simulink model "YMBOX_Control_Core"  (R2024b)
settings: Solver=FixedStepDiscrete  StartTime=0.0  StopTime=3  RelTol=1e-3
PreLoadFcn:
  | run(fullfile(fileparts(get_param(bdroot,'FileName')), 'YMBOX_Deluxe_init.m'));
InitFcn:
  | YMBOX_InitializeModel('core',bdroot);
model workspace (MAT data in the model file):
  KuMDAS_ObserverBuildVariant : Simulink.Parameter (value not decoded)
undefined symbols (not defined in the file or in its folder): CeMDSM_DrvModeIfStart_enum, CeMDSM_DrvModeSpdSens_enum, CeMDSM_DrvModeSpdSmo_enum, CeMDSM_DrvModeTrq_enum, Cf_CONTROL_TASK_TIME_S, KbMDAS_SmoDeadTimeCompEnable_flg, KbMDSA_ActiveInverterCompEnable_flg, KbMDSA_UnifiedVoltageLimitEnable_flg, KbMDSP_DCBusVoltReportFilterEnable_flg, KbMDTM_DAxisPriorityInFW_flg, KbMDTM_FieldWeakeningEnable_flg, KbMDTM_FinalIqAntiWindupEnable_flg, KbMDTM_SensorlessFieldWeakeningEnable_flg, KbMDTM_TorquePriorityBelowBase_flg, KbMDTM_UnifiedConstraintEnable_flg, KfMDAS_ControlCountToElecRad_NULL, KfMDAS_IfAccel_rpms, KfMDAS_IfAlignTime_s, KfMDAS_IfBlendTime_s, KfMDAS_IfSwitchSpd_rpm, KfMDAS_NativeCountToMechRad_NULL, KfMDAS_ObserverExitRatio_NULL, KfMDAS_SlsCtrlPeriod_s, KfMDAS_SlsEAngleInit_rad, KfMDAS_SlsElecSpdMax_rads, KfMDAS_SlsElecSpdMin_rads, KfMDAS_SlsTwoPi_rad, KfMDAS_SmoAngleOffset_rad, KfMDAS_SmoCurrentZohCoefA_NULL, KfMDAS_SmoCurrentZohCoefB_AperV, KfMDAS_SmoDeadTimeCurrentBoundary_A, KfMDAS_SmoDeadTimeDuty_NULL, KfMDAS_SmoDeadTimePolarity_NULL, KfMDAS_SmoDeviceDrop_V, KfMDAS_SmoEmfLpfCoefA_NULL, KfMDAS_SmoEmfLpfCoefB_NULL, KfMDAS_SmoEmfLpfInvPole_s, KfMDAS_SmoErrBoundaryMax_A, KfMDAS_SmoErrBoundarySpan_A, KfMDAS_SmoGainSchedAlpha_NULL, KfMDAS_SmoGainSchedAngleComp_rad, KfMDAS_SmoGainSchedEmfLow_V, KfMDAS_SmoGainSchedInvSpan_PerV, KfMDAS_SmoLdMinusLq_H, KfMDAS_SmoPllKiTs_NULL, KfMDAS_SmoPllKp_NULL, KfMDAS_SmoPllMinEmf_V, KfMDAS_SmoPllSpeedLpfAlpha_NULL, KfMDAS_SmoSlideGainMin_V, KfMDAS_SmoSlideGainSpan_V, KfMDAS_SmoSwitchSpd_rpm, KfMDAS_SmoTotalDelay_s, KfMDCC_DqSoftwareOverCurrentThreshold_A, KfMDCC_PiKcTsId_NULL, KfMDCC_PiKcTsIq_NULL, KfMDCC_PiKiTsId_NULL, KfMDCC_PiKiTsIq_NULL, KfMDCC_PiKpValueId_NULL, KfMDCC_PiKpValueIq_NULL, KfMDCC_PwmFreq_Hz ... (+84)
libraries: YMBOX_SharedMath_Lib x11, spsabctoAlphaBetaZeroLib x1
(part 2 of 8)

== system YMBOX_Control_Core/MDSP ==
  MINP_outputs : Inport  OutDataTypeStr=Bus: MINP_output
  MDSA_outputs : Inport  Port=2  OutDataTypeStr=Bus: MDSA_output
  trig_MDSP_ControlTask : TriggerPort  TriggerType=function-call  VariantControl=(inherit)
  DCBusCurrentFilterState : UnitDelay  InitialCondition=single(0)  SampleTime=-1
  DCBusCurrentInvalidHold : Switch  Threshold=0.5
  DCBusCurrentMean4 : MATLABSystem  System=dsp.simulink.MovingAverage  Method=Sliding window  ForgettingFactorPort=off  SpecifyWindowLength=on  WindowLength=KfMDSP_DCBusCurAvgWindow_cnt  OverlapLength=KfMDSP_DCBusCurAvgWindow_cnt-1  AllowArbitraryInputLength=off  ForgettingFactor=0.9  SimulateUsing=Code generation
      mask Type: dsp.simulink.MovingAverage
      mask Display: disp(['Moving' char(10) 'Average']);
  DCBus_Current_Source_Variant : Subsystem  Variant=on
  DCBus_Voltage_Filter : Subsystem
  Direct_Input_Selector : BusSelector  OutputSignals=VMIN_Dir_UCurSenrCurDet_A,VMIN_Dir_VCurSenrCurDet_A,VMIN_Dir_WCurSenrCurDet_A,VMIN_Dir_UCurSenrCurErr_NULL,VMIN_Dir_VCurSenrCurErr_NULL,VMIN_Dir_WCurSenrCurErr_NULL
  MDSP_Output_Bus : BusCreator  Inputs=13  OutDataTypeStr=Bus: MDSP_output  NonVirtualBus=on
      settings: InheritFromInputs=off
  MINP_Input_Selector : BusSelector  OutputSignals=Direct_Output,VuMINP_ResolverPositionRaw_NULL,VfMINP_DCBusVoltRaw_V
  MINP_Input_Selector1 : BusSelector  OutputSignals=VfMINP_DCBusCurPhysical_A
  PhaseSampleErrorAny : Logic  Operator=OR  Inputs=3
  PhaseSamplesValid : Logic  Operator=NOT  Inputs=1
  Phase_Current_Conditioning : Subsystem
  Previous_PWM_Selector : BusSelector  OutputSignals=VfMDSA_PwmDutyCyclePhaseU_NULL,VfMDSA_PwmDutyCyclePhaseV_NULL,VfMDSA_PwmDutyCyclePhaseW_NULL
  Resolver_Processing : Subsystem
  MDSP_outputs : Outport  OutDataTypeStr=Bus: MDSP_output
  wires:
  Direct_Input_Selector/2 -> DCBus_Current_Source_Variant/6(phaseV_A), Phase_Current_Conditioning/2(phaseV_A)  "<VMIN_Dir_VCurSenrCurDet_A>"
  Previous_PWM_Selector/2 -> DCBus_Current_Source_Variant/3(dutyV_NULL)  "<VfMDSA_PwmDutyCyclePhaseV_NULL>"
  Resolver_Processing/1(Resolver_Output) -> MDSP_Output_Bus/2  "Resolver_Output"
  DCBus_Voltage_Filter/3(VfMDSP_DCBusVoltReport_V) -> MDSP_Output_Bus/6  "VfMDSP_DCBusVoltReport_V"
  MDSP_Output_Bus/1 -> MDSP_outputs/1  "MDSP_output"
  MINP_Input_Selector/3 -> DCBus_Voltage_Filter/1(VfMINP_DCBusVoltRaw_V)  "<VfMINP_DCBusVoltRaw_V>"
  MINP_Input_Selector/2 -> Resolver_Processing/1(VuMINP_ResolverPositionRaw_NULL)  "<VuMINP_ResolverPositionRaw_NULL>"
  Direct_Input_Selector/1 -> DCBus_Current_Source_Variant/5(phaseU_A), Phase_Current_Conditioning/1(phaseU_A)  "<VMIN_Dir_UCurSenrCurDet_A>"
  Previous_PWM_Selector/3 -> DCBus_Current_Source_Variant/4(dutyW_NULL)  "<VfMDSA_PwmDutyCyclePhaseW_NULL>"
  Direct_Input_Selector/3 -> Phase_Current_Conditioning/3(phaseW_A), DCBus_Current_Source_Variant/7(phaseW_A)  "<VMIN_Dir_WCurSenrCurDet_A>"
  Direct_Input_Selector/4 -> Phase_Current_Conditioning/4(phaseUError_flg), PhaseSampleErrorAny/1  "<VMIN_Dir_UCurSenrCurErr_NULL>"
  Direct_Input_Selector/5 -> Phase_Current_Conditioning/5(phaseVError_flg), PhaseSampleErrorAny/2  "<VMIN_Dir_VCurSenrCurErr_NULL>"
  Direct_Input_Selector/6 -> Phase_Current_Conditioning/6(phaseWError_flg), PhaseSampleErrorAny/3  "<VMIN_Dir_WCurSenrCurErr_NULL>"
  MDSA_outputs/1 -> Previous_PWM_Selector/1
  PhaseSampleErrorAny/1 -> PhaseSamplesValid/1
  Previous_PWM_Selector/1 -> DCBus_Current_Source_Variant/2(dutyU_NULL)  "<VfMDSA_PwmDutyCyclePhaseU_NULL>"
  DCBus_Current_Source_Variant/2(currentValid_flg) -> DCBusCurrentInvalidHold/2, [currentValid_flg]  "VbMDSP_DCBusCurValid_flg"
  PhaseSamplesValid/1 -> DCBus_Current_Source_Variant/8(phaseSampleValid_flg)
  DCBusCurrentMean4/1 -> DCBusCurrentFilterState/1, [currentFilterd_A]  "VfMDSP_DCBusCur_Filtered_A"
  DCBus_Voltage_Filter/1(VfMDSP_DCBusVoltCtrl_V) -> MDSP_Output_Bus/4  "VfMDSP_DCBusVoltCtrl_V"
  DCBus_Voltage_Filter/2(VfMDSP_DCBusVoltRaw_V) -> MDSP_Output_Bus/5  "VfMDSP_DCBusVoltRaw_V"
  DCBus_Voltage_Filter/4(VbMDSP_DCBusVoltValid_flg) -> MDSP_Output_Bus/7  "VbMDSP_DCBusVoltValid_flg"
  DCBus_Current_Source_Variant/1(currentRaw_A) -> [currentRaw_A], DCBusCurrentInvalidHold/1  "VfMDSP_DCBusCurRaw_A"
  DCBusCurrentFilterState/1 -> DCBusCurrentInvalidHold/3
  DCBusCurrentInvalidHold/1 -> DCBusCurrentMean4/1
  MINP_Input_Selector/1 -> [DirectOutput]  "<Direct_Output>"
  [DirectOutput] -> Direct_Input_Selector/1
  [DirectOutput] -> MDSP_Output_Bus/1  "Direct_Output"
  [MINP_outputs] -> MINP_Input_Selector1/1
  MINP_outputs/1 -> [MINP_outputs]
  [MINP_outputs] -> MINP_Input_Selector/1
  MINP_Input_Selector1/1 -> DCBus_Current_Source_Variant/1(physicalCurrent_A)  "<VfMINP_DCBusCurPhysical_A>"
  [currentFilterd_A] -> MDSP_Output_Bus/3
  [currentValid_flg] -> MDSP_Output_Bus/9
  [currentRaw_A] -> MDSP_Output_Bus/8
  DCBus_Current_Source_Variant/3(sourceEnum) -> [sourceEnum]  "VuMDSP_DCBusCurSource_enum"
  [sourceEnum] -> MDSP_Output_Bus/10
  Phase_Current_Conditioning/1(VfMDSP_PhaseUCurrentCtrl_A) -> MDSP_Output_Bus/11  "VfMDSP_PhaseUCurrentCtrl_A"
  Phase_Current_Conditioning/2(VfMDSP_PhaseVCurrentCtrl_A) -> MDSP_Output_Bus/12  "VfMDSP_PhaseVCurrentCtrl_A"
  Phase_Current_Conditioning/3(VfMDSP_PhaseWCurrentCtrl_A) -> MDSP_Output_Bus/13  "VfMDSP_PhaseWCurrentCtrl_A"

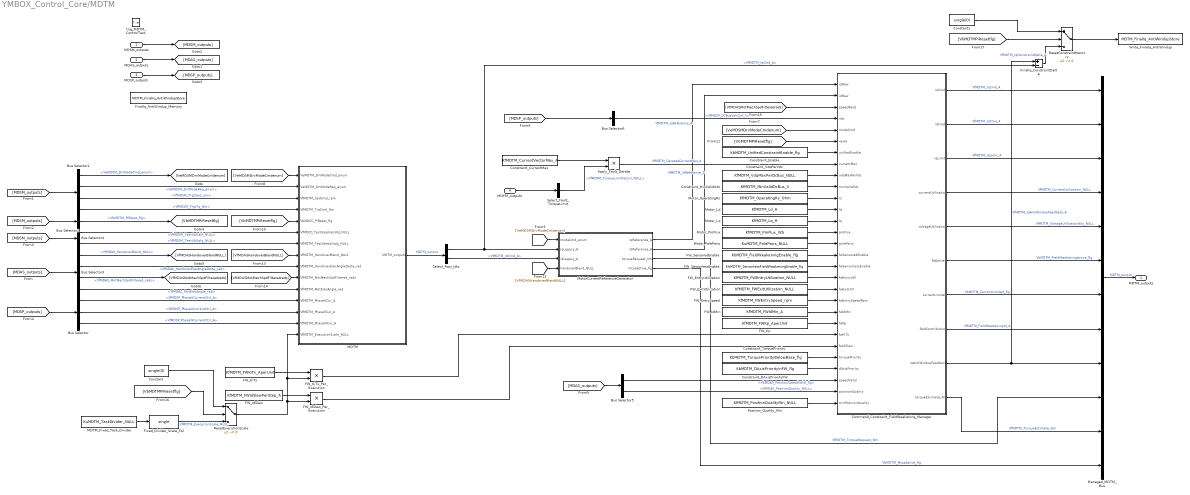
== system YMBOX_Control_Core/MDTM ==
  MDSM_outputs : Inport
  MDAS_outputs : Inport  Port=2
  MDSP_outputs : Inport  Port=3
  MDFM_outputs : Inport  Port=4
  trig_MDTM_ControlTask : TriggerPort  TriggerType=function-call  VariantControl=(inherit)
  Apply_Fault_Derate : Product  Inputs=**
  Bus Selector : BusSelector  OutputSignals=VfMDSP_PhaseUCurrentCtrl_A,VfMDSP_PhaseVCurrentCtrl_A,VfMDSP_PhaseWCurrentCtrl_A
  Bus Selector1 : BusSelector  OutputSignals=VeMDSM_DrvModeCmd_enum,VeMDSM_DrvModeReq_enum,VfMDSM_TrgtSpd_rpm,VfMDSM_TrgtTq_Nm
  Bus Selector2 : BusSelector  OutputSignals=VbMDTM_PiReset_flg
  Bus Selector3 : BusSelector  OutputSignals=VfMDAS_HandoverBlend_NULL,VfMDAS_HandoverElecAngleDelta_rad,VfMDAS_MotMechSpdFiltered_rads,VfMDAS_MotElecAngle_rad
  Bus Selector4 : BusSelector  OutputSignals=VfMDSM_TestUaUdId_NULL,VfMDSM_TestUbUqIq_NULL
  Bus Selector5 : BusSelector  OutputSignals=VbMDAS_PositionSpeedValid_flg,VfMDAS_PositionQuality_NULL
  Bus Selector6 : BusSelector  OutputSignals=VfMDSP_DCBusVoltCtrl_V
  Command_Constraint_FieldWeakening_Manager : Subsystem  Description=Modular final current-command constraint, field-weakening, utilization, torque-estimation, and anti-windup manager.
  Constant : Constant  Value=single(0)  OutDataTypeStr=single
  Constant1 : Constant  Value=single(0)  OutDataTypeStr=single
  Constraint_CurrentMax : Constant  Value=KfMDTM_CurrentVectorMax_A
  Constraint_DAxisPriorityFW : Constant  Value=KbMDTM_DAxisPriorityInFW_flg
  Constraint_Enable : Constant  Value=KbMDTM_UnifiedConstraintEnable_flg
  Constraint_MinValidVdc : Constant  Value=KfMDTM_MinValidDcBus_V
  Constraint_TorquePriority : Constant  Value=KbMDTM_TorquePriorityBelowBase_flg
  Constraint_VdqPerVdc : Constant  Value=KfMDTM_VdqMaxPerDcBus_NULL
  FW_EntrySpeed : Constant  Value=KfMDTM_FWEntrySpeed_rpm
  FW_EntryUtilization : Constant  Value=KfMDTM_FWEntryUtilization_NULL
  FW_ExitUtilization : Constant  Value=KfMDTM_FWExitUtilization_NULL
  FW_IdMin : Constant  Value=KfMDTM_FWIdMin_A
  FW_IdSlew : Constant  Value=KfMDTM_FWIdSlewPerStep_A
  FW_IdSlew_Per_Execution : Product  Inputs=**
  FW_KiTs : Constant  Value=KfMDTM_FWKiTs_AperUnit
  FW_KiTs_Per_Execution : Product  Inputs=**
  FW_Kp : Constant  Value=KfMDTM_FWKp_AperUnit
  FW_SensoredEnable : Constant  Value=KbMDTM_FieldWeakeningEnable_flg
  FW_SensorlessEnable : Constant  Value=KbMDTM_SensorlessFieldWeakeningEnable_flg
  FinalIq_AntiWindup_Memory : DataStoreMemory  DataStoreName=MDTM_FinalIq_AntiWindupStore  InitialValue=single(0)  ShowAdditionalParam=off  OutDataTypeStr=single
  FinalIq_ConstraintDelta : Sum  Inputs=+-
  Fixed_Divider_Scale_f32 : DataTypeConversion  OutDataTypeStr=single
  MDTM : Subsystem  Variant=on
      settings: AttributesFormatString=PRODUCT BUILD VARIANT\n0 SENSORED | 1 SMO
  MDTM_Fixed_Task_Divider : Constant  Value=KuMDTM_TaskDivider_NULL  OutDataTypeStr=uint16
  Managed_MDTM_Bus : BusCreator  Inputs=12  OutDataTypeStr=Bus: MDTM_output
  MotorCurrentReferenceGenerator : Subsystem  Variant=on
  Motor_Ld : Constant  Value=KfMDTM_Ld_H
  Motor_Lq : Constant  Value=KfMDTM_Lq_H
  Motor_OperatingRs : Constant  Value=KfMDTM_OperatingRs_Ohm
  Motor_PmFlux : Constant  Value=KfMDTM_PmFlux_Wb
  Motor_PolePairs : Constant  Value=KuMDTM_PolePairs_NULL
  Position_Quality_Min : Constant  Value=KfMDTM_PositionQualityMin_NULL
  ResetConstraintMemory : Switch  Criteria=u2 ~= 0
  ResetExecutionScale : Switch  Criteria=u2 ~= 0
  Select_Fault_TorqueLimit : BusSelector  OutputSignals=VfMDFM_TorqueLimitFactor_NULL
  Select_Raw_IdIq : BusSelector  OutputSignals=VfMDTM_IqCmd_A,VfMDTM_IdCmd_A
  Write_FinalIq_AntiWindup : DataStoreWrite  DataStoreName=MDTM_FinalIq_AntiWindupStore  IndexOptions=Index vector (dialog)  Indices=1  OutputSizes=1
  MDTM_outputs : Outport  OutDataTypeStr=Bus: MDTM_output
  wires:
  [MDSM_outputs] -> Bus Selector2/1
  MDSP_outputs/1 -> [MDSP_outputs]
  [MDSM_outputs] -> Bus Selector1/1
  [MDSM_outputs] -> Bus Selector4/1
  MDAS_outputs/1 -> [MDAS_outputs]
  [MDAS_outputs] -> Bus Selector3/1
  [MDSP_outputs] -> Bus Selector/1
  FW_ExitUtilization/1 -> Command_Constraint_FieldWeakening_Manager/19(fwExitUtil)
  MDSM_outputs/1 -> [MDSM_outputs]
  FW_IdSlew_Per_Execution/1 -> Command_Constraint_FieldWeakening_Manager/24(fwIdSlew)
  MDTM_Fixed_Task_Divider/1 -> Fixed_Divider_Scale_f32/1
  MDTM/1(MDTM_outputs) -> Select_Raw_IdIq/1  "MDTM_output"
  Bus Selector1/2 -> MDTM/2(VeMDTM_DrvModeReq_enum)  "<VeMDSM_DrvModeReq_enum>"
  Bus Selector1/4 -> MDTM/4(VfMDTM_TrqCmd_Nm)  "<VfMDSM_TrgtTq_Nm>"
  Bus Selector1/3 -> MDTM/3(VfMDTM_SpdCmd_rpm)  "<VfMDSM_TrgtSpd_rpm>"
  Bus Selector4/1 -> MDTM/6(VfMDCC_TestUalphaUdId_NULL)  "<VfMDSM_TestUaUdId_NULL>"
  Bus Selector4/2 -> MDTM/7(VfMDTM_TestUbetaUqIq_NULL)  "<VfMDSM_TestUbUqIq_NULL>"
  Bus Selector3/2 -> MDTM/9(VfMDTM_HandoverElecAngleDelta_rad)  "<VfMDAS_HandoverElecAngleDelta_rad>"
  Bus Selector3/4 -> MDTM/11(VfMDTM_MotElecAngle_rad)  "<VfMDAS_MotElecAngle_rad>"
  FW_KiTs_Per_Execution/1 -> Command_Constraint_FieldWeakening_Manager/23(fwKiTs)
  Bus Selector/1 -> MDTM/12(VfMDTM_PhaseUCur_A)  "<VfMDSP_PhaseUCurrentCtrl_A>"
  FW_Kp/1 -> Command_Constraint_FieldWeakening_Manager/22(fwKp)
  Bus Selector/3 -> MDTM/14(VfMDTM_PhaseWCur_A)  "<VfMDSP_PhaseWCurrentCtrl_A>"
  Bus Selector/2 -> MDTM/13(VfMDTM_PhaseVCur_A)  "<VfMDSP_PhaseVCurrentCtrl_A>"
  FW_KiTs/1 -> FW_KiTs_Per_Execution/1
  Motor_PolePairs/1 -> Command_Constraint_FieldWeakening_Manager/15(polePairs)
  Fixed_Divider_Scale_f32/1 -> ResetExecutionScale/3  "VfMDTM_ExecutionScale_NULL"
  Motor_PmFlux/1 -> Command_Constraint_FieldWeakening_Manager/14(pmFlux)
  FW_IdSlew/1 -> FW_IdSlew_Per_Execution/1
  MDFM_outputs/1 -> Select_Fault_TorqueLimit/1
  [MDSP_outputs] -> Bus Selector6/1
  Constraint_CurrentMax/1 -> Apply_Fault_Derate/1
  Select_Raw_IdIq/2 -> MotorCurrentReferenceGenerator/3(idLegacy_A)  "<VfMDTM_IdCmd_A>"
  Select_Raw_IdIq/1 -> FinalIq_ConstraintDelta/2, MotorCurrentReferenceGenerator/2(iqLegacy_A)  "<VfMDTM_IqCmd_A>"
  Constraint_MinValidVdc/1 -> Command_Constraint_FieldWeakening_Manager/10(minValidVdc)
  Select_Fault_TorqueLimit/1 -> Apply_Fault_Derate/2  "<VfMDFM_TorqueLimitFactor_NULL>"
  [MDAS_outputs] -> Bus Selector5/1
  Bus Selector6/1 -> Command_Constraint_FieldWeakening_Manager/4(vdc)  "<VfMDSP_DCBusVoltCtrl_V>"
  Apply_Fault_Derate/1 -> Command_Constraint_FieldWeakening_Manager/8(currentMax)  "VfMDTM_DeratedCurrentMax_A"
  Constraint_Enable/1 -> Command_Constraint_FieldWeakening_Manager/7(unifiedEnable)
  Motor_Ld/1 -> Command_Constraint_FieldWeakening_Manager/12(ld)
  Constraint_VdqPerVdc/1 -> Command_Constraint_FieldWeakening_Manager/9(vdqMaxPerVdc)
  Motor_OperatingRs/1 -> Command_Constraint_FieldWeakening_Manager/11(rs)
  Motor_Lq/1 -> Command_Constraint_FieldWeakening_Manager/13(lq)
  FW_SensoredEnable/1 -> Command_Constraint_FieldWeakening_Manager/16(fwSensoredEnable)
  MotorCurrentReferenceGenerator/1(iqReference_A) -> Command_Constraint_FieldWeakening_Manager/1(iqRaw)  "VfMDTM_IqReference_A"
  MotorCurrentReferenceGenerator/3(torqueRequest_Nm) -> Managed_MDTM_Bus/10  "VfMDTM_TorqueRequest_Nm"
  FinalIq_ConstraintDelta/1 -> ResetConstraintMemory/3  "VfMDTM_IqConstraintDelta_A"
  MotorCurrentReferenceGenerator/2(idReference_A) -> Command_Constraint_FieldWeakening_Manager/2(idRaw)  "VfMDTM_IdReference_A"
  MotorCurrentReferenceGenerator/4(mtpaActive_flg) -> Managed_MDTM_Bus/12  "VbMDTM_MtpaActive_flg"
  FW_SensorlessEnable/1 -> Command_Constraint_FieldWeakening_Manager/17(fwSensorlessEnable)
  FW_EntryUtilization/1 -> Command_Constraint_FieldWeakening_Manager/18(fwEntryUtil)
  FW_EntrySpeed/1 -> Command_Constraint_FieldWeakening_Manager/20(fwEntrySpeedRpm)
  FW_IdMin/1 -> Command_Constraint_FieldWeakening_Manager/21(fwIdMin)
  Command_Constraint_FieldWeakening_Manager/2(idCmd) -> Managed_MDTM_Bus/2  "VfMDTM_IdCmd_A"
  Command_Constraint_FieldWeakening_Manager/1(iqCmd) -> Managed_MDTM_Bus/1  "VfMDTM_IqCmd_A"
  Bus Selector5/2 -> Command_Constraint_FieldWeakening_Manager/28(positionQuality)  "<VfMDAS_PositionQuality_NULL>"
  Constraint_TorquePriority/1 -> Command_Constraint_FieldWeakening_Manager/25(torquePriority)
  Constraint_DAxisPriorityFW/1 -> Command_Constraint_FieldWeakening_Manager/26(dAxisPriority)
  Bus Selector5/1 -> Command_Constraint_FieldWeakening_Manager/27(speedValid)  "<VbMDAS_PositionSpeedValid_flg>"
  Position_Quality_Min/1 -> Command_Constraint_FieldWeakening_Manager/29(minPositionQuality)
  Command_Constraint_FieldWeakening_Manager/3(iqLimit) -> Managed_MDTM_Bus/3  "VfMDTM_IqLimit_A"
  Command_Constraint_FieldWeakening_Manager/4(currentUtilization) -> Managed_MDTM_Bus/4  "VfMDTM_CurrentUtilization_NULL"
  Command_Constraint_FieldWeakening_Manager/5(voltageUtilization) -> Managed_MDTM_Bus/5  "VfMDTM_VoltageUtilizationEst_NULL"
  Command_Constraint_FieldWeakening_Manager/6(fwActive) -> Managed_MDTM_Bus/6  "VbMDTM_FieldWeakeningActive_flg"
  Command_Constraint_FieldWeakening_Manager/7(currentLimited) -> Managed_MDTM_Bus/7  "VbMDTM_CurrentLimited_flg"
  Command_Constraint_FieldWeakening_Manager/8(fwIdContribution) -> Managed_MDTM_Bus/8  "VfMDTM_FieldWeakeningId_A"
  Command_Constraint_FieldWeakening_Manager/9(iqAntiWindupFeedback) -> Managed_MDTM_Bus/9, FinalIq_ConstraintDelta/1  "VfMDTM_IqAntiWindupFeedback_A"
  Command_Constraint_FieldWeakening_Manager/10(torqueEstimate_Nm) -> Managed_MDTM_Bus/11  "VfMDTM_TorqueEstimate_Nm"
  Managed_MDTM_Bus/1 -> MDTM_outputs/1  "MDTM_output"
  Bus Selector1/1 -> [VeMDSMDrvModeCmdenum]  "<VeMDSM_DrvModeCmd_enum>"
  [VeMDSMDrvModeCmdenum] -> Command_Constraint_FieldWeakening_Manager/5(modeCmd)
  [VeMDSMDrvModeCmdenum] -> MDTM/1(VeMDTM_DrvModeCmd_enum)
  [VeMDSMDrvModeCmdenum] -> MotorCurrentReferenceGenerator/1(modeCmd_enum)
  Bus Selector2/1 -> [VbMDTMPiResetflg]  "<VbMDTM_PiReset_flg>"
  [VbMDTMPiResetflg] -> MDTM/5(VbMDCC_PiReset_flg)
  [VbMDTMPiResetflg] -> Command_Constraint_FieldWeakening_Manager/6(reset)
  Bus Selector3/1 -> [VfMDASHandoverBlendNULL]  "<VfMDAS_HandoverBlend_NULL>"
  [VfMDASHandoverBlendNULL] -> MotorCurrentReferenceGenerator/4(handoverBlend_NULL)
  [VfMDASHandoverBlendNULL] -> MDTM/8(VfMDTM_HandoverBlend_NULL)
  Bus Selector3/3 -> [VfMDASMotMechSpdFilteredrads]  "<VfMDAS_MotMechSpdFiltered_rads>"
  [VfMDASMotMechSpdFilteredrads] -> MDTM/10(VfMDTM_MotMechSpdFiltered_rads)
  [VfMDASMotMechSpdFilteredrads] -> Command_Constraint_FieldWeakening_Manager/3(speedRads)
  Constant/1 -> ResetExecutionScale/1
  ResetConstraintMemory/1 -> Write_FinalIq_AntiWindup/1
  ResetExecutionScale/1 -> MDTM/15(VfMDTM_ExecutionScale_NULL), FW_KiTs_Per_Execution/2, FW_IdSlew_Per_Execution/2
  [VbMDTMPiResetflg] -> ResetExecutionScale/2
  Constant1/1 -> ResetConstraintMemory/1
  [VbMDTMPiResetflg] -> ResetConstraintMemory/2

== system YMBOX_Control_Core/MDAS/IF_Startup_Internal ==
  note: 1) Add Subsystem or Model blocks as valid variant choices.
      | 2) You cannot connect blocks at this level. At simulation, connectivity is automatically
      | determined, based on the active variant and port name matching.
  VeMDAS_DrvModeCmd_enum : Inport
  VeMDAS_DrvModeReq_enum : Inport  Port=2
  VfMDAS_TargetSpd_rpm : Inport  Port=3
  VfMDAS_SmoElecAngle_rad : Inport  Port=4
  VfMDAS_SmoElecSpd_rads : Inport  Port=5
  VfMDAS_SmoEmfMag_V : Inport  Port=6
  VfMDAS_SmoPllPhaseErr_NULL : Inport  Port=7
  IF_Startup_SMO : Subsystem  TreatAsAtomicUnit=on  VariantControl=KuMDAS_ObserverBuildVariant == 1
      settings: AttributesFormatString=PRODUCT SMO STARTUP\n16 I/F -> 17 SMO
  IF_Startup_SensoredOnly : Subsystem  TreatAsAtomicUnit=on  VariantControl=KuMDAS_ObserverBuildVariant == 0
      settings: AttributesFormatString=|
      | SENSORED ONLY
      | I/F startup and observer qualification omitted
  VfMDAS_IfMechSpd_rads : Outport
  VfMDAS_IfMechSpdAbs_rads : Outport  Port=2
  VfMDAS_IfElecAngle_rad : Outport  Port=3
  VfMDAS_SmoMechSpd_rads : Outport  Port=4
  VfMDAS_SmoMechSpdAbs_rads : Outport  Port=5
  VbMDAS_SmoReady_flg : Outport  Port=6
  VfMDAS_SmoAlignedElecAngle_rad : Outport  Port=7
  VfMDAS_HandoverBlend_NULL : Outport  Port=8
  VfMDAS_HandoverElecAngleDelta_rad : Outport  Port=9

== system YMBOX_Control_Core/MDAS/MDAS_DriveModeRoute_Variant ==
  note: 1) Add Subsystem or Model blocks as valid variant choices.
      | 2) You cannot connect blocks at this level. At simulation, connectivity is automatically
      | determined, based on the active variant and port name matching.
  <VeMDSM_DrvModeCmd_enum> : Inport
  <VuMDSP_MotMechAngleRaw_NULL> : Inport  Port=2
  VfMDAS_IfMechSpdAbs_rads : Inport  Port=3
  VfMDAS_IfMechSpd_rads : Inport  Port=4
  VfMDAS_SmoMechSpdAbs_rads : Inport  Port=5
  VfMDAS_SmoMechSpd_rads : Inport  Port=6
  VfMDAS_IfElecAngle_rad : Inport  Port=7
  VfMDAS_SmoAlignedElecAngle_rad : Inport  Port=8
  MDAS_Route_SMO : Subsystem  VariantControl=KuMDAS_ObserverBuildVariant == 1
      settings: AttributesFormatString=PRODUCT ROUTE\n1..5 SENSORED | 16 I/F | 17 SMO
  MDAS_Route_SensoredOnly : Subsystem  VariantControl=KuMDAS_ObserverBuildVariant == 0
      settings: AttributesFormatString=|
      | SENSORED ONLY
      | Resolver angle and speed calculation only
  VfMDAS_MotMechSpdFilteredAbs_rads : Outport
  VfMDAS_MotMechSpdFiltered_rads : Outport  Port=2
  VfMDAS_SelectedElecAngle_rad : Outport  Port=3

== system YMBOX_Control_Core/MDAS/Sensorless_FluxMRAS ==
  MDSP_outputs : Inport
  MDSA_outputs : Inport  Port=2
  MDSM_outputs : Inport  Port=3
  Observer_Variant0_SensoredOnly : Subsystem  VariantControl=KuMDAS_ObserverBuildVariant == 0
      settings: AttributesFormatString=PRODUCT VARIANT 0: SENSORED ONLY
  Observer_Variant1_SMO : Subsystem  TreatAsAtomicUnit=on  VariantControl=KuMDAS_ObserverBuildVariant == 1
      settings: AttributesFormatString=PRODUCT VARIANT 1: SMO ONLY
  VfMDAS_SmoElecAngle_rad : Outport
  VfMDAS_SmoElecSpd_rads : Outport  Port=2
  VfMDAS_SmoEmfMag_V : Outport  Port=3
  VfMDAS_SmoPllPhaseErr_NULL : Outport  Port=4

== system YMBOX_Control_Core/MDCC/MDCC_Subsystem ==
  VeMDCC_DrvModeCmd_enum : Inport
  VfMDCC_MotElecAngle_rad : Inport  Port=2
  VfMDCC_DCurCmd_A : Inport  Port=3
  VfMDCC_QCurCmd_A : Inport  Port=4
  VfMDCC_MotMechSpdFiltered_rads : Inport  Port=5
  VfMDCC_UCur_A : Inport  Port=6
  VfMDCC_VCur_A : Inport  Port=7
  VfMDCC_WCur_A : Inport  Port=8
  VfMDCC_TestUalphaUdId_NULL : Inport  Port=9
  VfMDCC_TestUbetaUqIq_NULL : Inport  Port=10
  VbMDCC_PiReset_flg : Inport  Port=11
  VuMDCC_FFEnable_enum : Inport  Port=12
  VfMDCC_k_effective_NULL : Inport  Port=13
  Clarke : Subsystem  RTWFcnName=vPwm_MDCC_Clarke  RTWFileName=MDCC
      settings: RTWSystemCode=Nonreusable function  RTWFcnNameOpts=User specified  RTWFileNameOpts=User specified  RTWMemSecFuncExecute=icache
  Constant2 : Constant  Value=KfMDCC_PiKpValueId_NULL
  Constant3 : Constant  Value=KfMDCC_PiKpValueIq_NULL
  DqSoftwareOverCurrent_Diagnostic : Subsystem
  DqSoftwareOverCurrent_PreviousTick : UnitDelay  InitialCondition=false  SampleTime=-1
  ElecAngle_SinCos_Adapter : Subsystem  RTWFcnName=vPwm_MDCC_LookUpEAngleCosSin  RTWFileName=MDCC
      settings: RTWSystemCode=Nonreusable function  RTWFcnNameOpts=User specified  RTWFileNameOpts=User specified  RTWMemSecFuncExecute=icache
  Park : Subsystem  RTWFcnName=vPwm_MDCC_Park  RTWFileName=MDCC
      settings: RTWSystemCode=Nonreusable function  RTWFcnNameOpts=User specified  RTWFileNameOpts=User specified  RTWMemSecFuncExecute=icache
  UdUqCalc : Subsystem  RTWFcnName=vPwm_MDCC_UdUqCalc  RTWFileName=MDCC
      settings: RTWSystemCode=Nonreusable function  RTWFcnNameOpts=User specified  RTWFileNameOpts=User specified  RTWMemSecFuncExecute=icache
  VfMDCC_VoltD_V : Outport
  VfMDCC_VoltQ_V : Outport  Port=2
  VbMDCC_DqSoftwareOverCurrent_flg : Outport  Port=3
  VfMDCC_DCur_A : Outport  Port=4
  VfMDCC_QCur_A : Outport  Port=5
  VfMDCC_EAngleCos_NULL : Outport  Port=6
  VfMDCC_EAngleSin_NULL : Outport  Port=7
  wires:
  VfMDCC_k_effective_NULL/1 -> UdUqCalc/13(VfMDCC_k_effective_NULL)  "VfMDCC_k_effective_NULL"
  VuMDCC_FFEnable_enum/1 -> UdUqCalc/12(VuMDCC_FFEnable_enum)
  VbMDCC_PiReset_flg/1 -> UdUqCalc/11(VbMDCC_PiReset_flg)
  VfMDCC_TestUbetaUqIq_NULL/1 -> UdUqCalc/10(VfMDCC_TestUbetaUqIq_NULL)
  VfMDCC_TestUalphaUdId_NULL/1 -> UdUqCalc/9(VfMDCC_TestUalphaUdId_NULL)
  Clarke/2(VfMDCC_BetaCur_A) -> Park/2(VfMDCC_BetaCur_A)
  VfMDCC_WCur_A/1 -> Clarke/3(VfMDCC_WCur_A)
  VfMDCC_VCur_A/1 -> Clarke/2(VfMDCC_VCur_A)
  VfMDCC_UCur_A/1 -> Clarke/1(VfMDCC_UCur_A)
  Clarke/1(VfMDCC_AlphaCur_A) -> Park/1(VfMDCC_AlphaCur_A)
  Constant3/1 -> UdUqCalc/8(VfMDCC_PiKpValueIq_NULL)  "VfMDCC_PiKpValueIq_NULL"
  VfMDCC_MotMechSpdFiltered_rads/1 -> UdUqCalc/6(VfMDCC_MotMechSpdFiltered_rads)
  VfMDCC_QCurCmd_A/1 -> UdUqCalc/5(VfMDCC_QCurCmd_A)
  VfMDCC_DCurCmd_A/1 -> UdUqCalc/4(VfMDCC_DCurCmd_A)
  Park/2(VfMDCC_QCur_A) -> VfMDCC_QCur_A/1, DqSoftwareOverCurrent_Diagnostic/2(VfMDCC_QCur_A), UdUqCalc/3(VfMDCC_QCur_A)
  Park/1(VfMDCC_DCur_A) -> VfMDCC_DCur_A/1, DqSoftwareOverCurrent_Diagnostic/1(VfMDCC_DCur_A), UdUqCalc/2(VfMDCC_DCur_A)
  VeMDCC_DrvModeCmd_enum/1 -> UdUqCalc/1(VeMDCC_DrvModeCmd_enum)
  ElecAngle_SinCos_Adapter/2(VfMDCC_EAngleSin_NULL) -> VfMDCC_EAngleSin_NULL/1, Park/4(VfMDCC_EAngleSin_NULL)  "VfMDCC_EAngleSin_NULL"
  ElecAngle_SinCos_Adapter/1(VfMDCC_EAngleCos_NULL) -> VfMDCC_EAngleCos_NULL/1, Park/3(VfMDCC_EAngleCos_NULL)  "VfMDCC_EAngleCos_NULL"
  VfMDCC_MotElecAngle_rad/1 -> ElecAngle_SinCos_Adapter/1(VfMDCC_MotElecAngle_rad)
  UdUqCalc/1(VfMDCC_VoltD_V) -> VfMDCC_VoltD_V/1  "VfMDCC_VoltD_V"
  UdUqCalc/2(VfMDCC_VoltQ_V) -> VfMDCC_VoltQ_V/1  "VfMDCC_VoltQ_V"
  Constant2/1 -> UdUqCalc/7(VfMDCC_PiKpValueId_NULL)  "VfMDCC_PiKpValueId_NULL"
  DqSoftwareOverCurrent_Diagnostic/1(VbMDCC_DqSoftwareOverCurrent_flg) -> DqSoftwareOverCurrent_PreviousTick/1  "VbMDCC_DqSoftwareOverCurrentRaw_flg"
  DqSoftwareOverCurrent_PreviousTick/1 -> VbMDCC_DqSoftwareOverCurrent_flg/1  "VbMDCC_DqSoftwareOverCurrent_flg"

== system YMBOX_Control_Core/MDFM/CommWatchdog ==
  aliveCounter : Inport
  enable : Inport  Port=2
  ArmOnEnable : Logic  Operator=OR  IconShape=distinctive
  CounterChanged : RelationalOperator  Operator=~=
  EnableArmedReset : Switch  Threshold=0.5
  EnableCountReset : Switch  Threshold=0.5
  False : Constant  Value=false  OutDataTypeStr=boolean
  FreshFrameReset : Switch  Threshold=0.5
  IncrementStaleCount : Sum  Inputs=|++
  LastAliveCounter : UnitDelay  InitialCondition=uint16(0)  SampleTime=-1
  One : Constant  Value=uint32(1)  OutDataTypeStr=uint32
  StaleCountBounded : Saturate  UpperLimit=KuMDFM_CommandTimeout_cnt  LowerLimit=0
  StaleCountState : UnitDelay  InitialCondition=uint32(0)  SampleTime=-1
  TimeoutAndArmed : Logic  IconShape=distinctive
  TimeoutReached : RelationalOperator  Operator=>
  TimeoutThreshold : Constant  Value=KuMDFM_CommandTimeout_cnt-1  OutDataTypeStr=uint32
  WatchdogArmedState : UnitDelay  InitialCondition=false  SampleTime=-1
  Zero : Constant  Value=uint32(0)  OutDataTypeStr=uint32
  commandTimeout : Outport
  staleCount : Outport  Port=2
  wires:
  IncrementStaleCount/1 -> StaleCountBounded/1
  StaleCountBounded/1 -> FreshFrameReset/3
  TimeoutReached/1 -> TimeoutAndArmed/1
  StaleCountState/1 -> IncrementStaleCount/1
  LastAliveCounter/1 -> CounterChanged/2
  EnableCountReset/1 -> staleCount/1, TimeoutReached/1, StaleCountState/1
  One/1 -> IncrementStaleCount/2
  enable/1 -> ArmOnEnable/2, EnableArmedReset/2, EnableCountReset/2
  CounterChanged/1 -> FreshFrameReset/2
  aliveCounter/1 -> CounterChanged/1, LastAliveCounter/1
  Zero/1 -> EnableCountReset/3, FreshFrameReset/1
  WatchdogArmedState/1 -> ArmOnEnable/1
  FreshFrameReset/1 -> EnableCountReset/1
  ArmOnEnable/1 -> EnableArmedReset/1
  TimeoutAndArmed/1 -> commandTimeout/1
  False/1 -> EnableArmedReset/3
  TimeoutThreshold/1 -> TimeoutReached/2
  EnableArmedReset/1 -> WatchdogArmedState/1, TimeoutAndArmed/2

== system YMBOX_Control_Core/MDFM/DCBus_Diagnostics ==
  MDSP_outputs : Inport  OutDataTypeStr=Bus: MDSP_output
  CurrentAboveHardMax : RelationalOperator  Operator=>
  CurrentBelowHardMin : RelationalOperator  Operator=<
  CurrentHardFault : Logic  Operator=OR  IconShape=distinctive
  CurrentHardMax : Constant  Value=KfMDFM_DCBusCurrentHardMax_A  OutDataTypeStr=single
  CurrentHardMin : Constant  Value=KfMDFM_DCBusCurrentHardMin_A  OutDataTypeStr=single
  CurrentSource_Copy : SignalConversion  OverrideOpt=off
  CurrentValid_Copy : SignalConversion  OverrideOpt=off
  RawCurrent_Copy : SignalConversion  OverrideOpt=off
  Select_DCBus_Data : BusSelector  OutputSignals=VfMDSP_DCBusCurRaw_A,VfMDSP_DCBusCur_Filtered_A,VbMDSP_DCBusCurValid_flg,VuMDSP_DCBusCurSource_enum,VfMDSP_DCBusVoltReport_V
  SoftCurrent_Copy : SignalConversion  OverrideOpt=off
  VoltageReport_Copy : SignalConversion  OverrideOpt=off
  currentRaw : Outport  OutDataTypeStr=single
  currentSoft : Outport  Port=2  OutDataTypeStr=single
  currentValid : Outport  Port=3  OutDataTypeStr=boolean
  currentHardFault : Outport  Port=4  OutDataTypeStr=boolean
  currentSource : Outport  Port=5  OutDataTypeStr=uint8
  voltageReport : Outport  Port=6  OutDataTypeStr=single
  wires:
  MDSP_outputs/1 -> Select_DCBus_Data/1
  CurrentHardMax/1 -> CurrentAboveHardMax/2
  Select_DCBus_Data/1 -> CurrentBelowHardMin/1, CurrentAboveHardMax/1, RawCurrent_Copy/1  "<VfMDSP_DCBusCurRaw_A>"
  Select_DCBus_Data/2 -> SoftCurrent_Copy/1  "<VfMDSP_DCBusCur_Filtered_A>"
  Select_DCBus_Data/3 -> CurrentValid_Copy/1  "<VbMDSP_DCBusCurValid_flg>"
  Select_DCBus_Data/4 -> CurrentSource_Copy/1  "<VuMDSP_DCBusCurSource_enum>"
  Select_DCBus_Data/5 -> VoltageReport_Copy/1  "<VfMDSP_DCBusVoltReport_V>"
  CurrentHardMin/1 -> CurrentBelowHardMin/2
  RawCurrent_Copy/1 -> currentRaw/1
  SoftCurrent_Copy/1 -> currentSoft/1
  CurrentValid_Copy/1 -> currentValid/1
  CurrentSource_Copy/1 -> currentSource/1
  CurrentAboveHardMax/1 -> CurrentHardFault/1
  CurrentBelowHardMin/1 -> CurrentHardFault/2
  VoltageReport_Copy/1 -> voltageReport/1
  CurrentHardFault/1 -> currentHardFault/1

== system YMBOX_Control_Core/MDFM/PhaseSWOC_Qualifier ==
  iu : Inport
  iv : Inport  Port=2
  iw : Inport  Port=3
  enable : Inport  Port=4
  iuError : Inport  Port=5  OutDataTypeStr=boolean
  ivError : Inport  Port=6  OutDataTypeStr=boolean
  iwError : Inport  Port=7  OutDataTypeStr=boolean
  AbsPhaseU : Abs
  AbsPhaseV : Abs
  AbsPhaseW : Abs
  Constant : Constant  Value=single(0)  OutDataTypeStr=single
  CountDecrement : Sum  Inputs=+-  OutDataTypeStr=int32  AccumDataTypeStr=int32
  CountDirectionSelect : Switch  Threshold=0.5
  CountIncrement : Sum  OutDataTypeStr=uint16  SaturateOnIntegerOverflow=on
  DecrementBounded : Saturate  UpperLimit=int32(65535)  LowerLimit=int32(0)  OutDataTypeStr=uint16
  EnableReset : Switch  Threshold=0.5
  IncrementBounded : Saturate  UpperLimit=KuMDFM_PhaseSoftwareOverCurrentConfirm_cnt  LowerLimit=uint16(0)  OutDataTypeStr=uint16
  MaxPhaseCurrent : MinMax  Function=max  Inputs=3
  One : Constant  Value=uint16(1)  OutDataTypeStr=uint16
  OverCurrentCountState : UnitDelay  InitialCondition=uint16(0)  SampleTime=-1
  PhaseCurrentLimitExceeded : RelationalOperator  Operator=>
  PhaseSoftwareOverCurrentConfirmCountMinusOne : Constant  Value=KuMDFM_PhaseSoftwareOverCurrentConfirm_cnt-uint16(1)  OutDataTypeStr=uint16
  PhaseSoftwareOverCurrentLimit : Constant  Value=KfMDFM_PhaseSoftwareOverCurrent_A
  PhaseSoftwareOverCurrentQualified : RelationalOperator  Operator=>
  Sel0 : Switch  Criteria=u2 ~= 0
  Sel1 : Switch  Criteria=u2 ~= 0
  Sel2 : Switch  Criteria=u2 ~= 0
  Zero : Constant  Value=uint16(0)  OutDataTypeStr=uint16
  phaseSoftwareOverCurrent : Outport
  wires:
  PhaseSoftwareOverCurrentLimit/1 -> PhaseCurrentLimitExceeded/2
  OverCurrentCountState/1 -> CountDecrement/1, CountIncrement/1
  iu/1 -> AbsPhaseU/1
  AbsPhaseV/1 -> Sel1/3
  iv/1 -> AbsPhaseV/1
  PhaseSoftwareOverCurrentQualified/1 -> phaseSoftwareOverCurrent/1
  iw/1 -> AbsPhaseW/1
  enable/1 -> EnableReset/2
  AbsPhaseU/1 -> Sel0/3
  One/1 -> CountIncrement/2, CountDecrement/2
  PhaseSoftwareOverCurrentConfirmCountMinusOne/1 -> PhaseSoftwareOverCurrentQualified/2
  AbsPhaseW/1 -> Sel2/3
  CountIncrement/1 -> IncrementBounded/1
  MaxPhaseCurrent/1 -> PhaseCurrentLimitExceeded/1
  CountDecrement/1 -> DecrementBounded/1
  CountDirectionSelect/1 -> EnableReset/1
  IncrementBounded/1 -> CountDirectionSelect/1
  PhaseCurrentLimitExceeded/1 -> CountDirectionSelect/2
  DecrementBounded/1 -> CountDirectionSelect/3
  Zero/1 -> EnableReset/3
  EnableReset/1 -> OverCurrentCountState/1, PhaseSoftwareOverCurrentQualified/1
  iuError/1 -> Sel0/2
  Sel0/1 -> MaxPhaseCurrent/1
  ivError/1 -> Sel1/2
  Sel1/1 -> MaxPhaseCurrent/2
  iwError/1 -> Sel2/2
  Sel2/1 -> MaxPhaseCurrent/3
  Constant/1 -> Sel1/1, Sel2/1, Sel0/1

== system YMBOX_Control_Core/MDFM/VoltageQual ==
  vdc : Inport
  enable : Inport  Port=2
  OverAreaBounded : Saturate  UpperLimit=2*KfMDFM_VoltageViolationArea_Vs  LowerLimit=0
  OverAreaCandidate : Sum
  OverAreaState : UnitDelay  SampleTime=-1
  OverAreaStep : Gain  Gain=Cf_CONTROL_TASK_TIME_S
  OverDeltaSelect : Switch  Threshold=0.5
  OverPositiveOnly : Saturate  UpperLimit=inf  LowerLimit=0
  OverViolationActive : RelationalOperator  Operator=>
  OverVoltageExcess : Sum  Inputs=+-
  OverVoltageLimit : Constant  Value=KfMDFM_DcBusOverVoltage_V
  OverVoltageQualified : RelationalOperator  Operator=>
  RecoveryStep : Constant  Value=-KfMDFM_VoltageRecoveryRate_V*Cf_CONTROL_TASK_TIME_S  OutDataTypeStr=single
  UnderAreaBounded : Saturate  UpperLimit=2*KfMDFM_VoltageViolationArea_Vs  LowerLimit=0
  UnderAreaCandidate : Sum
  UnderAreaState : UnitDelay  SampleTime=-1
  UnderAreaStep : Gain  Gain=Cf_CONTROL_TASK_TIME_S
  UnderDeltaSelect : Switch  Threshold=0.5
  UnderEnableReset : Switch  Threshold=0.5
  UnderPositiveOnly : Saturate  UpperLimit=inf  LowerLimit=0
  UnderViolationActive : RelationalOperator  Operator=>
  UnderVoltageExcess : Sum  Inputs=+-
  UnderVoltageLimit : Constant  Value=KfMDFM_DcBusUnderVoltage_V
  UnderVoltageQualified : Logic  IconShape=distinctive  AllPortsSameDT=off  OutDataTypeStr=boolean
  UnderVoltageQualifiedRaw : RelationalOperator  Operator=>
  ViolationAreaLimit : Constant  Value=KfMDFM_VoltageViolationArea_Vs
  Zero : Constant  Value=single(0)  OutDataTypeStr=single
  dcOverVoltage : Outport
  dcUnderVoltage : Outport  Port=2
  wires:
  OverVoltageLimit/1 -> OverVoltageExcess/2
  UnderPositiveOnly/1 -> UnderViolationActive/1, UnderAreaStep/1
  OverAreaCandidate/1 -> OverAreaBounded/1
  UnderVoltageExcess/1 -> UnderPositiveOnly/1
  vdc/1 -> UnderVoltageExcess/2, OverVoltageExcess/1
  OverPositiveOnly/1 -> OverViolationActive/1, OverAreaStep/1
  Zero/1 -> OverViolationActive/2, UnderViolationActive/2, UnderEnableReset/3
  OverVoltageExcess/1 -> OverPositiveOnly/1
  UnderVoltageLimit/1 -> UnderVoltageExcess/1
  enable/1 -> UnderVoltageQualified/2, UnderEnableReset/2
  UnderVoltageQualified/1 -> dcUnderVoltage/1
  OverAreaStep/1 -> OverDeltaSelect/1
  OverViolationActive/1 -> OverDeltaSelect/2
  OverDeltaSelect/1 -> OverAreaCandidate/2
  UnderAreaStep/1 -> UnderDeltaSelect/1
  RecoveryStep/1 -> OverDeltaSelect/3, UnderDeltaSelect/3
  OverVoltageQualified/1 -> dcOverVoltage/1
  OverAreaBounded/1 -> OverAreaState/1, OverVoltageQualified/1
  UnderViolationActive/1 -> UnderDeltaSelect/2
  UnderEnableReset/1 -> UnderAreaState/1
  OverAreaState/1 -> OverAreaCandidate/1
  UnderDeltaSelect/1 -> UnderAreaCandidate/1
  UnderAreaState/1 -> UnderAreaCandidate/2
  UnderAreaCandidate/1 -> UnderAreaBounded/1
  UnderAreaBounded/1 -> UnderVoltageQualifiedRaw/1, UnderEnableReset/1
  ViolationAreaLimit/1 -> UnderVoltageQualifiedRaw/2, OverVoltageQualified/2
  UnderVoltageQualifiedRaw/1 -> UnderVoltageQualified/1

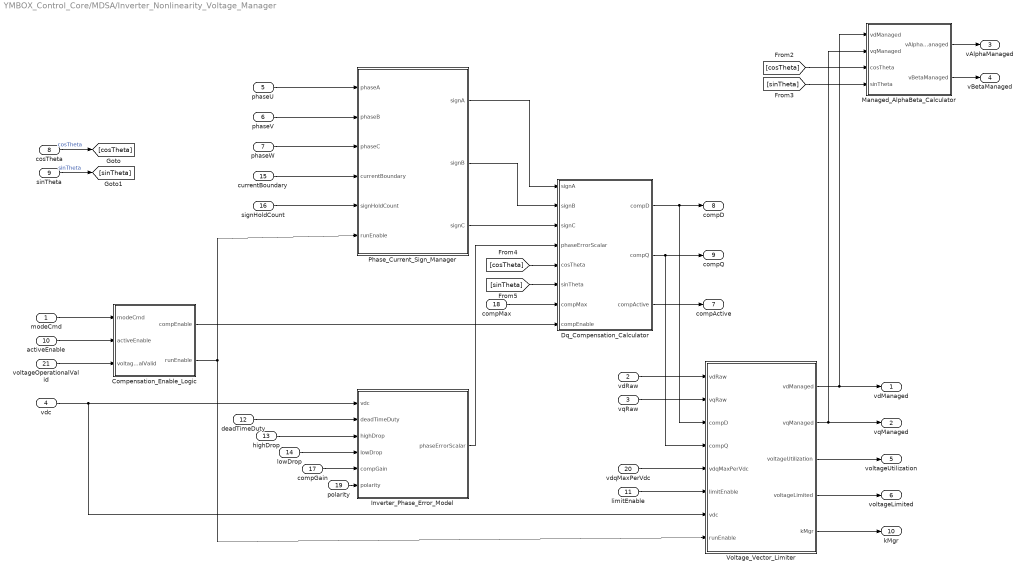
== system YMBOX_Control_Core/MDSA/Inverter_Nonlinearity_Voltage_Manager ==
  modeCmd : Inport
  vdRaw : Inport  Port=2
  vqRaw : Inport  Port=3
  vdc : Inport  Port=4
  phaseU : Inport  Port=5  OutDataTypeStr=single
  phaseV : Inport  Port=6  OutDataTypeStr=single
  phaseW : Inport  Port=7  OutDataTypeStr=single
  cosTheta : Inport  Port=8  OutDataTypeStr=single
  sinTheta : Inport  Port=9  OutDataTypeStr=single
  activeEnable : Inport  Port=10
  limitEnable : Inport  Port=11
  deadTimeDuty : Inport  Port=12
  highDrop : Inport  Port=13
  lowDrop : Inport  Port=14
  currentBoundary : Inport  Port=15
  signHoldCount : Inport  Port=16
  compGain : Inport  Port=17
  compMax : Inport  Port=18
  polarity : Inport  Port=19
  vdqMaxPerVdc : Inport  Port=20
  voltageOperationalValid : Inport  Port=21  OutDataTypeStr=boolean
  Compensation_Enable_Logic : Subsystem
  Dq_Compensation_Calculator : Subsystem
  Inverter_Phase_Error_Model : Subsystem
  Managed_AlphaBeta_Calculator : Subsystem
  Phase_Current_Sign_Manager : Subsystem
  Voltage_Vector_Limiter : Subsystem
  vdManaged : Outport
  vqManaged : Outport  Port=2
  vAlphaManaged : Outport  Port=3
  vBetaManaged : Outport  Port=4
  voltageUtilization : Outport  Port=5
  voltageLimited : Outport  Port=6
  compActive : Outport  Port=7
  compD : Outport  Port=8
  compQ : Outport  Port=9
  kMgr : Outport  Port=10
  wires:
  vdc/1 -> Inverter_Phase_Error_Model/1(vdc), Voltage_Vector_Limiter/7(vdc)
  Dq_Compensation_Calculator/3(compActive) -> compActive/1
  modeCmd/1 -> Compensation_Enable_Logic/1(modeCmd)
  limitEnable/1 -> Voltage_Vector_Limiter/6(limitEnable)
  activeEnable/1 -> Compensation_Enable_Logic/2(activeEnable)
  vdqMaxPerVdc/1 -> Voltage_Vector_Limiter/5(vdqMaxPerVdc)
  lowDrop/1 -> Inverter_Phase_Error_Model/4(lowDrop)
  currentBoundary/1 -> Phase_Current_Sign_Manager/4(currentBoundary)
  highDrop/1 -> Inverter_Phase_Error_Model/3(highDrop)
  deadTimeDuty/1 -> Inverter_Phase_Error_Model/2(deadTimeDuty)
  Dq_Compensation_Calculator/2(compQ) -> Voltage_Vector_Limiter/4(compQ), compQ/1
  compGain/1 -> Inverter_Phase_Error_Model/5(compGain)
  signHoldCount/1 -> Phase_Current_Sign_Manager/5(signHoldCount)
  Compensation_Enable_Logic/1(compEnable) -> Dq_Compensation_Calculator/8(compEnable)
  Compensation_Enable_Logic/2(runEnable) -> Phase_Current_Sign_Manager/6(runEnable), Voltage_Vector_Limiter/8(runEnable)
  compMax/1 -> Dq_Compensation_Calculator/7(compMax)
  polarity/1 -> Inverter_Phase_Error_Model/6(polarity)
  Phase_Current_Sign_Manager/1(signA) -> Dq_Compensation_Calculator/1(signA)
  Phase_Current_Sign_Manager/2(signB) -> Dq_Compensation_Calculator/2(signB)
  Phase_Current_Sign_Manager/3(signC) -> Dq_Compensation_Calculator/3(signC)
  Inverter_Phase_Error_Model/1(phaseErrorScalar) -> Dq_Compensation_Calculator/4(phaseErrorScalar)
  Dq_Compensation_Calculator/1(compD) -> Voltage_Vector_Limiter/3(compD), compD/1
  vqRaw/1 -> Voltage_Vector_Limiter/2(vqRaw)
  vdRaw/1 -> Voltage_Vector_Limiter/1(vdRaw)
  Voltage_Vector_Limiter/1(vdManaged) -> vdManaged/1, Managed_AlphaBeta_Calculator/1(vdManaged)
  Voltage_Vector_Limiter/2(vqManaged) -> vqManaged/1, Managed_AlphaBeta_Calculator/2(vqManaged)
  Voltage_Vector_Limiter/3(voltageUtilization) -> voltageUtilization/1
  Voltage_Vector_Limiter/4(voltageLimited) -> voltageLimited/1
  Managed_AlphaBeta_Calculator/1(vAlphaManaged) -> vAlphaManaged/1
  Managed_AlphaBeta_Calculator/2(vBetaManaged) -> vBetaManaged/1
  cosTheta/1 -> [cosTheta]  "cosTheta"
  sinTheta/1 -> [sinTheta]  "sinTheta"
  [sinTheta] -> Managed_AlphaBeta_Calculator/4(sinTheta)
  [cosTheta] -> Managed_AlphaBeta_Calculator/3(cosTheta)
  [cosTheta] -> Dq_Compensation_Calculator/5(cosTheta)
  [sinTheta] -> Dq_Compensation_Calculator/6(sinTheta)
  Voltage_Vector_Limiter/5(kMgr) -> kMgr/1
  phaseU/1 -> Phase_Current_Sign_Manager/1(phaseA)
  phaseV/1 -> Phase_Current_Sign_Manager/2(phaseB)
  phaseW/1 -> Phase_Current_Sign_Manager/3(phaseC)
  voltageOperationalValid/1 -> Compensation_Enable_Logic/3(voltageOperationalValid)

== system YMBOX_Control_Core/MDSA/MDSA_Subsystem ==
  VeMDSA_DrvModeCmd_enum : Inport
  VfMDSA_VoltD_V : Inport  Port=2
  VfMDSA_VoltQ_V : Inport  Port=3
  VfMDSA_MotElecAngle_rad : Inport  Port=4
  VfMDSA_MotElecSpd_rads : Inport  Port=5
  VfMDSA_DCBusVolt_V : Inport  Port=6
  VfMDSA_PwmFreq_Hz : Inport  Port=7
  VfMDSA_TestUalphaUdId_NULL : Inport  Port=8
  VfMDSA_TestUbetaUqIq_NULL : Inport  Port=9
  VbMDFM_VoltageOperationalValid_flg : Inport  Port=10  OutDataTypeStr=boolean
  PwmOutput : Subsystem  RTWFcnName=vPwm_MDSA_PwmOutput  RTWFileName=MDSA
      settings: RTWSystemCode=Nonreusable function  RTWFcnNameOpts=User specified  RTWFileNameOpts=User specified
  UalphaUbetaCalc : Subsystem  RTWFcnName=vPwm_MDSA_UalphaUbetaCalc  RTWFileName=MDSA
      settings: RTWSystemCode=Nonreusable function  RTWFcnNameOpts=User specified  RTWFileNameOpts=User specified
  VfMDSA_PwmDutyCyclePhaseU_NULL : Outport
  VfMDSA_PwmDutyCyclePhaseV_NULL : Outport  Port=2
  VfMDSA_PwmDutyCyclePhaseW_NULL : Outport  Port=3
  VfMDSA_k_svm_NULL : Outport  Port=4
  wires:
  PwmOutput/4(VfMDSA_k_svm_NULL) -> VfMDSA_k_svm_NULL/1
  VfMDSA_PwmFreq_Hz/1 -> UalphaUbetaCalc/6(VfMDSA_PwmFreq_Hz)
  VeMDSA_DrvModeCmd_enum/1 -> PwmOutput/1(VeMDSA_DrvModeCmd_enum), UalphaUbetaCalc/1(VeMDSA_DrvModeCmd_enum)
  VfMDSA_TestUbetaUqIq_NULL/1 -> UalphaUbetaCalc/8(VfMDSA_TestUbetaUqIq_NULL)
  PwmOutput/3(VfMDSA_PwmDutyCyclePhaseW_NULL) -> VfMDSA_PwmDutyCyclePhaseW_NULL/1
  PwmOutput/2(VfMDSA_PwmDutyCyclePhaseV_NULL) -> VfMDSA_PwmDutyCyclePhaseV_NULL/1
  PwmOutput/1(VfMDSA_PwmDutyCyclePhaseU_NULL) -> VfMDSA_PwmDutyCyclePhaseU_NULL/1
  VfMDSA_DCBusVolt_V/1 -> PwmOutput/4(VfMDSA_DCBusVolt_V)
  UalphaUbetaCalc/2(VfMDSA_VoltBeta_V) -> PwmOutput/3(VfMDSA_VoltBeta_V)
  UalphaUbetaCalc/1(VfMDSA_VoltAlpha_V) -> PwmOutput/2(VfMDSA_VoltAlpha_V)
  VfMDSA_TestUalphaUdId_NULL/1 -> UalphaUbetaCalc/7(VfMDSA_TestUalphaUdId_NULL)
  VfMDSA_MotElecSpd_rads/1 -> UalphaUbetaCalc/5(VfMDSA_MotElecSpd_rads)
  VfMDSA_MotElecAngle_rad/1 -> UalphaUbetaCalc/4(VfMDSA_MotElecAngle_rad)
  VfMDSA_VoltQ_V/1 -> UalphaUbetaCalc/3(VfMDSA_VoltQ_V)  "VfMDSA_VoltQ_V"
  VfMDSA_VoltD_V/1 -> UalphaUbetaCalc/2(VfMDSA_VoltD_V)  "VfMDSA_VoltD_V"
  VbMDFM_VoltageOperationalValid_flg/1 -> PwmOutput/5(VbMDFM_VoltageOperationalValid_flg)

== system YMBOX_Control_Core/MDSM/MDSM_ModeManager ==
  VeMDSM_DrvModeReq_enum : Inport
  VbMDSM_MCUEnb_flg : Inport  Port=2
  VbMDAS_SmoReady_flg : Inport  Port=3
  VfMDSM_TrgtSpd_rpm : Inport  Port=4
  MDSM_RouteConfig_Variant : Subsystem  Variant=on
      settings: AttributesFormatString=PRODUCT ROUTE VARIANT\n0 SENSORED | 1 I/F -> SMO
  MDSM_Supervisor_Variant : Subsystem  Variant=on
      settings: AttributesFormatString=PRODUCT BUILD VARIANT\n0 SENSORED | 1 SMO
  VeMDSM_DrvModeCmd_enum : Outport
  VbMDTM_PiReset_flg : Outport  Port=2
  VbMDCC_PiReset_flg : Outport  Port=3
  VuMDFM_FFEnable_enum : Outport  Port=4
  wires:
  VeMDSM_DrvModeReq_enum/1 -> MDSM_Supervisor_Variant/7(VeMDSM_DrvModeReq_enum), [RI_ModeReq]
  [RI_ModeReq] -> MDSM_RouteConfig_Variant/1(VeMDSM_DrvModeReq_enum)
  VbMDAS_SmoReady_flg/1 -> [RI_SmoReady]
  [RI_SmoReady] -> MDSM_RouteConfig_Variant/2(VbMDAS_SmoReady_flg)
  MDSM_RouteConfig_Variant/1(VbMDSM_RouteSupported_flg) -> [CFG_Supported]
  MDSM_RouteConfig_Variant/6(VeMDSM_Stage1Mode_enum) -> [CFG_Stage1Mode]
  MDSM_RouteConfig_Variant/2(VbMDSM_Stage1Ready_flg) -> [CFG_Stage1Ready]
  MDSM_RouteConfig_Variant/8(VfMDSM_Stage1SwitchSpd_rpm) -> [CFG_Stage1Switch]
  MDSM_RouteConfig_Variant/10(VuMDSM_Stage1Acquire_cnt) -> [CFG_Stage1Acquire]
  MDSM_RouteConfig_Variant/3(VbMDSM_Stage2Enable_flg) -> [CFG_Stage2Enable]
  MDSM_RouteConfig_Variant/7(VeMDSM_Stage2Mode_enum) -> [CFG_Stage2Mode]
  MDSM_RouteConfig_Variant/5(VbMDSM_Stage2Ready_flg) -> [CFG_Stage2Ready]
  MDSM_RouteConfig_Variant/9(VfMDSM_Stage2SwitchSpd_rpm) -> [CFG_Stage2Switch]
  MDSM_RouteConfig_Variant/4(VbMDSM_Stage2Fallback_flg) -> [CFG_Stage2Fallback]
  VbMDSM_MCUEnb_flg/1 -> MDSM_Supervisor_Variant/1(VbMDSM_MCUEnb_flg)
  [CFG_Supported] -> MDSM_Supervisor_Variant/2(VbMDSM_RouteSupported_flg)
  [CFG_Stage1Mode] -> MDSM_Supervisor_Variant/8(VeMDSM_Stage1Mode_enum)
  [CFG_Stage1Ready] -> MDSM_Supervisor_Variant/3(VbMDSM_Stage1Ready_flg)
  [CFG_Stage1Switch] -> MDSM_Supervisor_Variant/10(VfMDSM_Stage1SwitchSpd_rpm)
  [CFG_Stage1Acquire] -> MDSM_Supervisor_Variant/13(VuMDSM_Stage1Acquire_cnt)
  [CFG_Stage2Enable] -> MDSM_Supervisor_Variant/4(VbMDSM_Stage2Enable_flg)
  [CFG_Stage2Mode] -> MDSM_Supervisor_Variant/9(VeMDSM_Stage2Mode_enum)
  [CFG_Stage2Ready] -> MDSM_Supervisor_Variant/6(VbMDSM_Stage2Ready_flg)
  [CFG_Stage2Switch] -> MDSM_Supervisor_Variant/11(VfMDSM_Stage2SwitchSpd_rpm)
  [CFG_Stage2Fallback] -> MDSM_Supervisor_Variant/5(VbMDSM_Stage2Fallback_flg)
  VfMDSM_TrgtSpd_rpm/1 -> MDSM_Supervisor_Variant/12(VfMDSM_TrgtSpd_rpm)
  MDSM_Supervisor_Variant/3(VeMDSM_DrvModeCmd_enum) -> VeMDSM_DrvModeCmd_enum/1  "VeMDSM_DrvModeCmd_enum"
  MDSM_Supervisor_Variant/2(VbMDTM_PiReset_flg) -> VbMDTM_PiReset_flg/1  "VbMDTM_PiReset_flg"
  MDSM_Supervisor_Variant/1(VbMDCC_PiReset_flg) -> VbMDCC_PiReset_flg/1  "VbMDCC_PiReset_flg"
  MDSM_Supervisor_Variant/4(VuMDFM_FFEnable_enum) -> VuMDFM_FFEnable_enum/1  "VuMDFM_FFEnable_enum"

== system YMBOX_Control_Core/MDSP/DCBus_Current_Source_Variant ==
  note: 1) Add Subsystem or Model blocks as valid variant choices.
      | 2) You cannot connect blocks at this level. At simulation, connectivity is automatically
      | determined, based on the active variant and port name matching.
  physicalCurrent_A : Inport  OutDataTypeStr=single
  dutyU_NULL : Inport  Port=2  OutDataTypeStr=single
  dutyV_NULL : Inport  Port=3  OutDataTypeStr=single
  dutyW_NULL : Inport  Port=4  OutDataTypeStr=single
  phaseU_A : Inport  Port=5  OutDataTypeStr=single
  phaseV_A : Inport  Port=6  OutDataTypeStr=single
  phaseW_A : Inport  Port=7  OutDataTypeStr=single
  phaseSampleValid_flg : Inport  Port=8  OutDataTypeStr=boolean
  EstimatedFromFOC : Subsystem  VariantControl=KuMDSP_DCBusCurSource_enum == 1
  PhysicalSensor : Subsystem  VariantControl=KuMDSP_DCBusCurSource_enum == 0
  currentRaw_A : Outport  OutDataTypeStr=single
  currentValid_flg : Outport  Port=2  OutDataTypeStr=boolean
  sourceEnum : Outport  Port=3  OutDataTypeStr=uint8

== system YMBOX_Control_Core/MDSP/DCBus_Voltage_Filter ==
  VfMINP_DCBusVoltRaw_V : Inport  OutDataTypeStr=single
  VdcAboveInitMin : RelationalOperator
  VdcAboveMin : RelationalOperator
  VdcAlpha : Gain  Gain=KfMDSP_DCBusVoltControlFilterAlpha_NULL
  VdcBelowMax : RelationalOperator  Operator=<=
  VdcErr : Sum  Inputs=+-
  VdcFirstValidInitialize : Switch  Threshold=0.5
  VdcInitEligible : Logic  IconShape=distinctive
  VdcInitMin : Constant  Value=KfMDSP_DCBusVoltInitMin_V
  VdcInitializationHold : Switch  Threshold=0.5
  VdcInitializedNext : Logic  Operator=OR  IconShape=distinctive
  VdcInitializedState : UnitDelay  InitialCondition=false  SampleTime=-1
  VdcInvalidHold : Switch  Threshold=0.5
  VdcPlausibleMax : Constant  Value=KfMDSP_DCBusVoltPlausibleMax_V
  VdcPlausibleMin : Constant  Value=KfMDSP_DCBusVoltPlausibleMin_V
  VdcRawValid : Logic  IconShape=distinctive
  VdcReportAlpha : Gain  Gain=KfMDSP_DCBusVoltReportFilterAlpha_NULL
  VdcReportErr : Sum  Inputs=-+
  VdcReportFilterEnable : Constant  Value=KbMDSP_DCBusVoltReportFilterEnable_flg
  VdcReportFilterSelect : Switch  Threshold=0.5
  VdcReportFirstValidInitialize : Switch  Threshold=0.5
  VdcReportInvalidHold : Switch  Threshold=0.5
  VdcReportState : UnitDelay  InitialCondition=single(0)  SampleTime=-1
  VdcReportUpdate : Sum
  VdcState : UnitDelay  InitialCondition=single(0)  SampleTime=-1
  VdcUpdate : Sum
  VfMDSP_DCBusVoltCtrl_V : Outport  OutDataTypeStr=single
  VfMDSP_DCBusVoltRaw_V : Outport  Port=2  OutDataTypeStr=single
  VfMDSP_DCBusVoltReport_V : Outport  Port=3  OutDataTypeStr=single
  VbMDSP_DCBusVoltValid_flg : Outport  Port=4  OutDataTypeStr=boolean
  wires:
  VfMINP_DCBusVoltRaw_V/1 -> VdcErr/1, VdcAboveInitMin/1, VdcBelowMax/1, VdcAboveMin/1, VdcFirstValidInitialize/3, VfMDSP_DCBusVoltRaw_V/1
  VdcPlausibleMin/1 -> VdcAboveMin/2
  VdcAboveMin/1 -> VdcRawValid/1
  VdcInvalidHold/1 -> VfMDSP_DCBusVoltCtrl_V/1, VdcState/1, VdcReportErr/2, VdcReportFilterSelect/3, VdcReportFirstValidInitialize/3
  VdcPlausibleMax/1 -> VdcBelowMax/2
  VdcInitMin/1 -> VdcAboveInitMin/2
  VdcRawValid/1 -> VdcInitEligible/2, VdcReportInvalidHold/2, VbMDSP_DCBusVoltValid_flg/1, VdcInvalidHold/2
  VdcReportFilterSelect/1 -> VfMDSP_DCBusVoltReport_V/1
  VdcBelowMax/1 -> VdcRawValid/2
  VdcReportAlpha/1 -> VdcReportUpdate/1
  VdcAboveInitMin/1 -> VdcInitEligible/1
  VdcUpdate/1 -> VdcFirstValidInitialize/1
  VdcInitEligible/1 -> VdcInitializedNext/2
  VdcInitializedState/1 -> VdcFirstValidInitialize/2, VdcInitializedNext/1, VdcReportFirstValidInitialize/2
  VdcState/1 -> VdcInvalidHold/3, VdcInitializationHold/3, VdcErr/2, VdcUpdate/2
  VdcFirstValidInitialize/1 -> VdcInitializationHold/1
  VdcReportFirstValidInitialize/1 -> VdcReportInvalidHold/1
  VdcInitializationHold/1 -> VdcInvalidHold/1
  VdcInitializedNext/1 -> VdcInitializationHold/2, VdcInitializedState/1
  VdcErr/1 -> VdcAlpha/1
  VdcAlpha/1 -> VdcUpdate/1
  VdcReportUpdate/1 -> VdcReportFirstValidInitialize/1
  VdcReportState/1 -> VdcReportErr/1, VdcReportInvalidHold/3, VdcReportUpdate/2
  VdcReportInvalidHold/1 -> VdcReportFilterSelect/1, VdcReportState/1
  VdcReportFilterEnable/1 -> VdcReportFilterSelect/2
  VdcReportErr/1 -> VdcReportAlpha/1
